simulink subsystem "Stewart_Platform"  (R2020a)
settings: Solver=VariableStepAuto  StartTime=0.0  StopTime=10.0  RelTol=1e-3
settings Model: Creator=thomas  LastModifiedBy=thomas

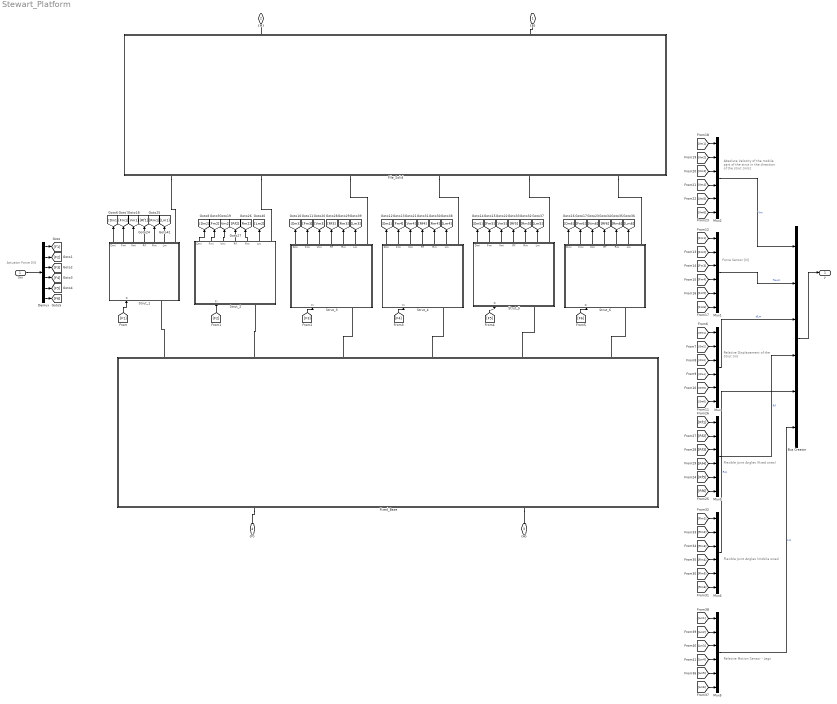
== system Stewart_Platform ==
  note: Flexible Joint Angles (fixed ones)
  note: Force Sensor [N]
  note: Relative Displacement
      | of the Strut [m]
  note: Absolute Velocity of the
      | mobile part of the strut in
      | the direction of the strut [m/s]
  note: Actuator Force [N]
  note: Flexible Joint Angles (mobile ones)
  note: Relative Motion Sensor - Legs
  tau : Inport
  Bus Creator : BusCreator  Inputs=6
  Demux : Demux  Outputs=6
  File_Solid : Subsystem  VariantControl=Choice  ReferencedSubsystem=Mobile_Platform
  Fixed_Base : Subsystem  VariantControl=stewart.platform_F.type == 2  ReferencedSubsystem=Fixed_Based
  Mux{,1..5} (6 alike) : Mux  Inputs=6
  Strut_1 : Subsystem
      mask init:
      | i=1;
  Strut_2 : Subsystem
      mask init:
      | i=2;
  Strut_3 : Subsystem
      mask init:
      | i=3;
  Strut_4 : Subsystem
      mask init:
      | i=4;
  Strut_5 : Subsystem
      mask init:
      | i=5;
  Strut_6 : Subsystem
      mask init:
      | i=6;
  "{B}" : PMIOPort  Side=Right
  "{M}" : PMIOPort  Port=2  Side=Right
  "{A}" : PMIOPort  Port=3  Side=Left
  "{F}" : PMIOPort  Port=4  Side=Left
  y : Outport
  wires:
  [Vm3] -> Mux2/3
  [F3] -> Strut_3/1(Fi)
  [F4] -> Strut_4/1(Fi)
  Strut_5/1(Dmi) -> [Dm5]
  [F1] -> Strut_1/1(Fi)
  Strut_1/2(Fmi) -> [Fm1]
  Demux/5 -> [F5]
  Demux/1 -> [F1]
  Demux/6 -> [F6]
  [Fm2] -> Mux1/2
  Strut_3/1(Dmi) -> [Dm3]
  Demux/3 -> [F3]
  [Fm4] -> Mux1/4
  [Vm2] -> Mux2/2
  [Dm4] -> Mux/4
  Strut_2/1(Dmi) -> [Dm2]
  Strut_6/2(Fmi) -> [Fm6]
  [Vm5] -> Mux2/5
  Strut_1/3(Vmi) -> [Vm1]
  Mux1/1 -> Bus Creator/2  "Taum"
  [Vm1] -> Mux2/1
  Demux/2 -> [F2]
  Mux/1 -> Bus Creator/3  "dLm"
  Strut_6/1(Dmi) -> [Dm6]
  [Dm5] -> Mux/5
  Strut_2/3(Vmi) -> [Vm2]
  [F2] -> Strut_2/1(Fi)
  [Fm6] -> Mux1/6
  Strut_4/1(Dmi) -> [Dm4]
  [Dm2] -> Mux/2
  Strut_6/3(Vmi) -> [Vm6]
  [F5] -> Strut_5/1(Fi)
  [Vm6] -> Mux2/6
  [Fm5] -> Mux1/5
  Strut_3/3(Vmi) -> [Vm3]
  Strut_5/2(Fmi) -> [Fm5]
  Strut_4/2(Fmi) -> [Fm4]
  Strut_5/3(Vmi) -> [Vm5]
  [Vm4] -> Mux2/4
  [F6] -> Strut_6/1(Fi)
  [Fm3] -> Mux1/3
  Mux2/1 -> Bus Creator/1  "Vm"
  [Dm3] -> Mux/3
  tau/1 -> Demux/1
  Strut_3/2(Fmi) -> [Fm3]
  Strut_1/1(Dmi) -> [Dm1]
  Demux/4 -> [F4]
  Strut_2/2(Fmi) -> [Fm2]
  [Dm6] -> Mux/6
  [Fm1] -> Mux1/1
  [Dm1] -> Mux/1
  Strut_4/3(Vmi) -> [Vm4]
  Bus Creator/1 -> y/1
  [Rf1] -> Mux3/1
  [Rf2] -> Mux3/2
  [Rf3] -> Mux3/3
  [Rf4] -> Mux3/4
  [Rf5] -> Mux3/5
  [Rf6] -> Mux3/6
  [Rm1] -> Mux4/1
  [Rm2] -> Mux4/2
  [Rm3] -> Mux4/3
  [Rm4] -> Mux4/4
  [Rm5] -> Mux4/5
  [Rm6] -> Mux4/6
  Mux3/1 -> Bus Creator/4  "Rf"
  Mux4/1 -> Bus Creator/5  "Rm"
  Strut_1/4(Rf) -> [Rf1]
  Strut_1/5(Rm) -> [Rm1]
  Strut_3/5(Rm) -> [Rm3]
  Strut_3/4(Rf) -> [Rf3]
  Strut_4/5(Rm) -> [Rm4]
  Strut_4/4(Rf) -> [Rf4]
  Strut_5/4(Rf) -> [Rf5]
  Strut_5/5(Rm) -> [Rm5]
  Strut_6/4(Rf) -> [Rf6]
  Strut_6/5(Rm) -> [Rm6]
  Strut_2/4(Rf) -> [Rf2]
  Strut_2/5(Rm) -> [Rm2]
  Strut_6/6(Lm) -> [Lm6]
  Strut_5/6(Lm) -> [Lm5]
  Strut_4/6(Lm) -> [Lm4]
  Strut_3/6(Lm) -> [Lm3]
  Strut_2/6(Lm) -> [Lm2]
  Strut_1/6(Lm) -> [Lm1]
  Mux5/1 -> Bus Creator/6  "Lm"
  [Lm6] -> Mux5/6
  [Lm5] -> Mux5/5
  [Lm4] -> Mux5/4
  [Lm3] -> Mux5/3
  [Lm2] -> Mux5/2
  [Lm1] -> Mux5/1
  connections:
  Fixed_Base/LConn1 -- "{F}"/RConn1
  Fixed_Base/LConn2 -- "{A}"/RConn1
  Fixed_Base/RConn1 -- Strut_1/LConn1
  Fixed_Base/RConn2 -- Strut_2/LConn1
  Fixed_Base/RConn3 -- Strut_3/LConn1
  Fixed_Base/RConn4 -- Strut_4/LConn1
  Fixed_Base/RConn5 -- Strut_5/LConn1
  Fixed_Base/RConn6 -- Strut_6/LConn1
  File_Solid/LConn1 -- Strut_1/RConn1
  File_Solid/LConn2 -- Strut_2/RConn1
  File_Solid/LConn3 -- Strut_3/RConn1
  File_Solid/LConn4 -- Strut_4/RConn1
  File_Solid/LConn5 -- Strut_5/RConn1
  File_Solid/LConn6 -- Strut_6/RConn1
  File_Solid/RConn1 -- "{M}"/RConn1
  File_Solid/RConn2 -- "{B}"/RConn1

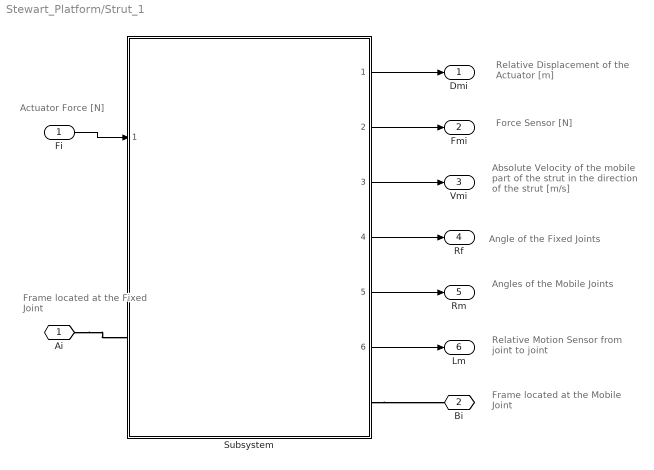
== system Stewart_Platform/Strut_1 ==
  note: Angle of the Fixed Joints
  note: Angles of the Mobile Joints
  note: Relative Motion Sensor
      | from joint to joint
  note: Frame located at
      | the Mobile Joint
  note: Actuator Force [N]
  note: Frame located at
      | the Fixed Joint
  note: Force Sensor [N]
  note: Relative Displacement
      | of the Actuator [m]
  note: Absolute Velocity of the
      | mobile part of the strut in
      | the direction of the strut [m/s]
  Fi : Inport
  Subsystem : Subsystem  VariantControl=with_sensors  ReferencedSubsystem=stewart_strut
  Ai : PMIOPort  Side=Left
  Bi : PMIOPort  Port=2  Side=Right
  Dmi : Outport
  Fmi : Outport  Port=2
  Vmi : Outport  Port=3
  Rf : Outport  Port=4
  Rm : Outport  Port=5
  Lm : Outport  Port=6
  wires:
  Subsystem/6 -> Lm/1
  Subsystem/5 -> Rm/1
  Subsystem/4 -> Rf/1
  Fi/1 -> Subsystem/1
  Subsystem/3 -> Vmi/1
  Subsystem/2 -> Fmi/1
  Subsystem/1 -> Dmi/1
  connections:
  Subsystem/RConn1 -- Bi/RConn1
  Ai/RConn1 -- Subsystem/LConn1

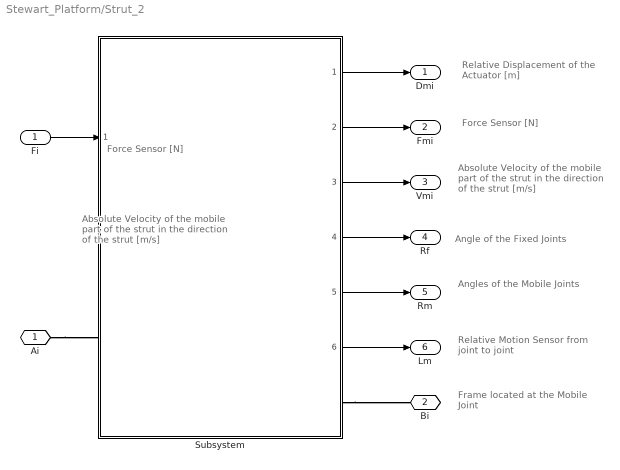
== system Stewart_Platform/Strut_2 ==
  note: Angles of the Mobile Joints
  note: Force Sensor [N]
  note: Angle of the Fixed Joints
  note: Relative Motion Sensor
      | from joint to joint
  note: Relative Displacement
      | of the Actuator [m]
  note: Frame located at
      | the Mobile Joint
  note: Absolute Velocity of the
      | mobile part of the strut in
      | the direction of the strut [m/s]
  note: Absolute Velocity of the
      | mobile part of the strut in
      | the direction of the strut [m/s]
  note: Force Sensor [N]
  Fi : Inport
  Subsystem : Subsystem  VariantControl=with_sensors  ReferencedSubsystem=stewart_strut
  Ai : PMIOPort  Side=Left
  Bi : PMIOPort  Port=2  Side=Right
  Dmi : Outport
  Fmi : Outport  Port=2
  Vmi : Outport  Port=3
  Rf : Outport  Port=4
  Rm : Outport  Port=5
  Lm : Outport  Port=6
  wires:
  Subsystem/4 -> Rf/1
  Subsystem/2 -> Fmi/1
  Subsystem/6 -> Lm/1
  Subsystem/5 -> Rm/1
  Subsystem/1 -> Dmi/1
  Subsystem/3 -> Vmi/1
  Fi/1 -> Subsystem/1
  connections:
  Subsystem/RConn1 -- Bi/RConn1
  Ai/RConn1 -- Subsystem/LConn1

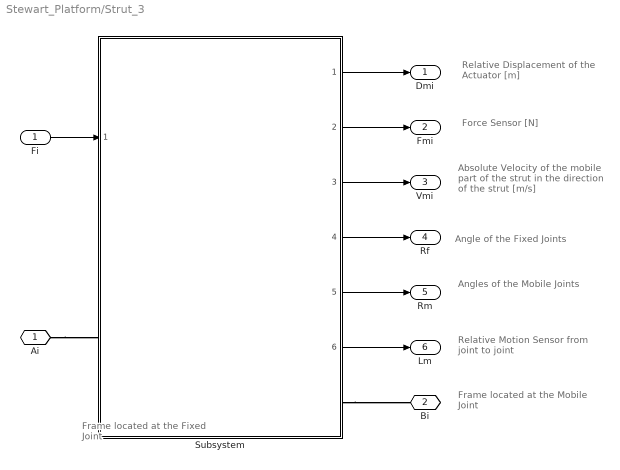
== system Stewart_Platform/Strut_3 ==
  note: Angles of the Mobile Joints
  note: Force Sensor [N]
  note: Angle of the Fixed Joints
  note: Relative Motion Sensor
      | from joint to joint
  note: Relative Displacement
      | of the Actuator [m]
  note: Frame located at
      | the Mobile Joint
  note: Absolute Velocity of the
      | mobile part of the strut in
      | the direction of the strut [m/s]
  note: Frame located at
      | the Fixed Joint
  Fi : Inport
  Subsystem : Subsystem  VariantControl=with_sensors  ReferencedSubsystem=stewart_strut
  Ai : PMIOPort  Side=Left
  Bi : PMIOPort  Port=2  Side=Right
  Dmi : Outport
  Fmi : Outport  Port=2
  Vmi : Outport  Port=3
  Rf : Outport  Port=4
  Rm : Outport  Port=5
  Lm : Outport  Port=6
  wires:
  Subsystem/4 -> Rf/1
  Subsystem/2 -> Fmi/1
  Subsystem/6 -> Lm/1
  Subsystem/5 -> Rm/1
  Subsystem/1 -> Dmi/1
  Subsystem/3 -> Vmi/1
  Fi/1 -> Subsystem/1
  connections:
  Subsystem/RConn1 -- Bi/RConn1
  Ai/RConn1 -- Subsystem/LConn1

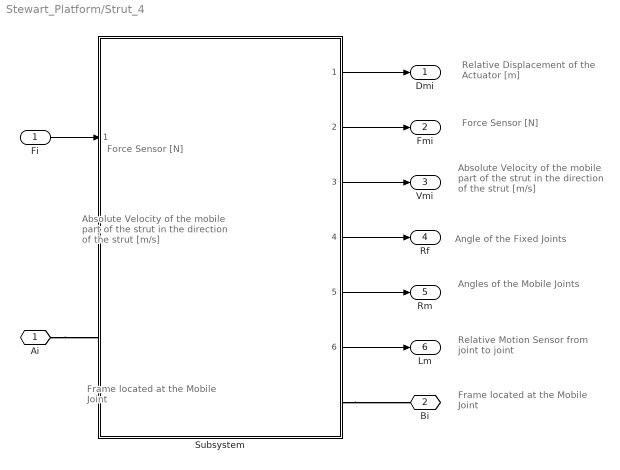
== system Stewart_Platform/Strut_4 ==
  note: Angles of the Mobile Joints
  note: Force Sensor [N]
  note: Angle of the Fixed Joints
  note: Relative Motion Sensor
      | from joint to joint
  note: Relative Displacement
      | of the Actuator [m]
  note: Frame located at
      | the Mobile Joint
  note: Absolute Velocity of the
      | mobile part of the strut in
      | the direction of the strut [m/s]
  note: Absolute Velocity of the
      | mobile part of the strut in
      | the direction of the strut [m/s]
  note: Force Sensor [N]
  note: Frame located at
      | the Mobile Joint
  Fi : Inport
  Subsystem : Subsystem  VariantControl=with_sensors  ReferencedSubsystem=stewart_strut
  Ai : PMIOPort  Side=Left
  Bi : PMIOPort  Port=2  Side=Right
  Dmi : Outport
  Fmi : Outport  Port=2
  Vmi : Outport  Port=3
  Rf : Outport  Port=4
  Rm : Outport  Port=5
  Lm : Outport  Port=6
  wires:
  Subsystem/4 -> Rf/1
  Subsystem/2 -> Fmi/1
  Subsystem/6 -> Lm/1
  Subsystem/5 -> Rm/1
  Subsystem/1 -> Dmi/1
  Subsystem/3 -> Vmi/1
  Fi/1 -> Subsystem/1
  connections:
  Subsystem/RConn1 -- Bi/RConn1
  Ai/RConn1 -- Subsystem/LConn1

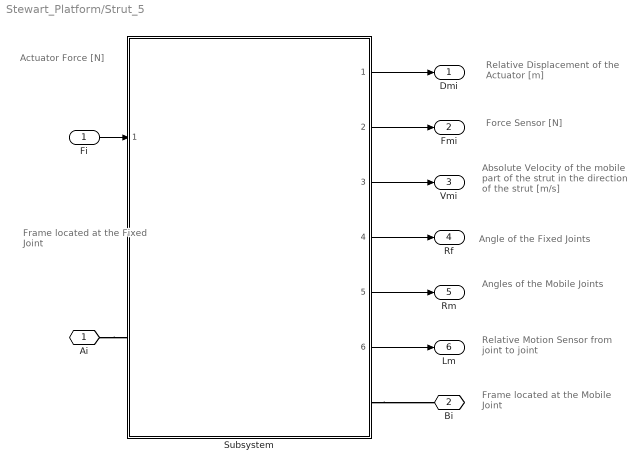
== system Stewart_Platform/Strut_5 ==
  note: Angles of the Mobile Joints
  note: Force Sensor [N]
  note: Angle of the Fixed Joints
  note: Relative Motion Sensor
      | from joint to joint
  note: Relative Displacement
      | of the Actuator [m]
  note: Frame located at
      | the Mobile Joint
  note: Absolute Velocity of the
      | mobile part of the strut in
      | the direction of the strut [m/s]
  note: Actuator Force [N]
  note: Frame located at
      | the Fixed Joint
  Fi : Inport
  Subsystem : Subsystem  VariantControl=with_sensors  ReferencedSubsystem=stewart_strut
  Ai : PMIOPort  Side=Left
  Bi : PMIOPort  Port=2  Side=Right
  Dmi : Outport
  Fmi : Outport  Port=2
  Vmi : Outport  Port=3
  Rf : Outport  Port=4
  Rm : Outport  Port=5
  Lm : Outport  Port=6
  wires:
  Subsystem/4 -> Rf/1
  Subsystem/2 -> Fmi/1
  Subsystem/6 -> Lm/1
  Subsystem/5 -> Rm/1
  Subsystem/1 -> Dmi/1
  Subsystem/3 -> Vmi/1
  Fi/1 -> Subsystem/1
  connections:
  Subsystem/RConn1 -- Bi/RConn1
  Ai/RConn1 -- Subsystem/LConn1

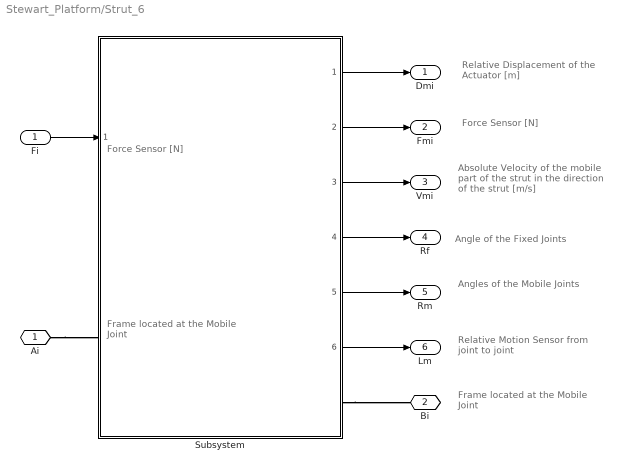
== system Stewart_Platform/Strut_6 ==
  note: Angles of the Mobile Joints
  note: Force Sensor [N]
  note: Angle of the Fixed Joints
  note: Relative Motion Sensor
      | from joint to joint
  note: Relative Displacement
      | of the Actuator [m]
  note: Frame located at
      | the Mobile Joint
  note: Absolute Velocity of the
      | mobile part of the strut in
      | the direction of the strut [m/s]
  note: Force Sensor [N]
  note: Frame located at
      | the Mobile Joint
  Fi : Inport
  Subsystem : Subsystem  VariantControl=with_sensors  ReferencedSubsystem=stewart_strut
  Ai : PMIOPort  Side=Left
  Bi : PMIOPort  Port=2  Side=Right
  Dmi : Outport
  Fmi : Outport  Port=2
  Vmi : Outport  Port=3
  Rf : Outport  Port=4
  Rm : Outport  Port=5
  Lm : Outport  Port=6
  wires:
  Subsystem/4 -> Rf/1
  Subsystem/2 -> Fmi/1
  Subsystem/6 -> Lm/1
  Subsystem/5 -> Rm/1
  Subsystem/1 -> Dmi/1
  Subsystem/3 -> Vmi/1
  Fi/1 -> Subsystem/1
  connections:
  Subsystem/RConn1 -- Bi/RConn1
  Ai/RConn1 -- Subsystem/LConn1
